simulink model "oc_exm_counter"  (Simulink 6.5)
settings: Solver=FixedStepDiscrete  StartTime=0.0  StopTime=10.0  FixedStep=0.001  RelTol=1e-3
libraries: dsPICdrivers x9
settings Model: Creator=Peter  LastModifiedBy=peter  ProdHWDeviceType=16-bit Generic
settings SolverCC: PositivePriorityOrder=on
settings OptimizationCC: OptimizeModelRefInitCode=on  LifeSpan=1
settings HardwareCC: ProdBitPerInt=16  ProdEndianess=LittleEndian  ProdWordSize=16  ProdHWDeviceType=16-bit Generic  TargetHWDeviceType=32-bit Generic
settings RTWCC: SystemTargetFile=dspic.tlc  TemplateMakefile=dspic_pic30_gcc.tmf  PostCodeGenCommand=dsPIC_Compile()  Description=Embedded Target for Microchip dsPIC (real-time)  ProcessScript=dspic_make_rtw_hook
settings CodeAppCC: IgnoreCustomStorageClasses=off
settings STFCustomTargetCC: TargetFcnLib=ansi_tfl_tmw.mat  GenFloatMathFcnCalls=ANSI_C  ModelReferenceCompliant=off  IncludeMdlTerminateFcn=off  CombineOutputUpdateFcns=on  SuppressErrorStatus=on  ERTCustomFileBanners=on  SupportContinuousTime=off  SupportNonInlinedSFcns=off  SystemTargetFile=dspic.tlc
settings ERTTargetCC: TargetFcnLib=ansi_tfl_tmw.mat  GenFloatMathFcnCalls=ANSI_C  ModelReferenceCompliant=off  IncludeMdlTerminateFcn=off  SuppressErrorStatus=on  InlinedParameterPlacement=NonHierarchical  ERTSrcFileBannerTemplate=dsPIC_code_template.cgt  ERTHdrFileBannerTemplate=dsPIC_code_template.cgt  ERTDataSrcFileTemplate=dsPIC_code_template.cgt  ERTDataHdrFileTemplate=dsPIC_code_template.cgt  ERTCustomFileTemplate=dsPIC_main.tlc
settings CustomProperty: DataType=string  Value=C:\MATLAB\R2006b\rtw\bin\win32\gmake

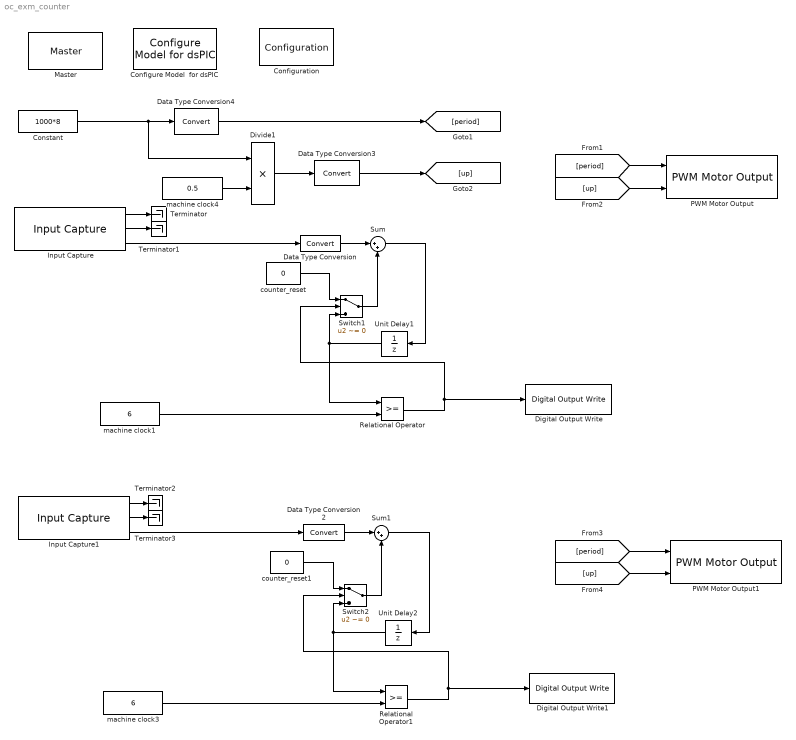
== system oc_exm_counter ==
  Configuration : dsPICdrivers/Configuration  SystemSampleTime=-1  double64=on
  Configure Model  for dsPIC : dsPICdrivers/Simulink Configuration/Configure Model  for dsPIC
  Constant : Constant  Value=1000*8  OutDataTypeMode=double  OutDataType=sfix(16)  ConRadixGroup=Use specified scaling  OutScaling=2^0  SampleTime=-1  FramePeriod=inf
  Data Type Conversion : DataTypeConversion  OutDataTypeMode=double
  Data Type Conversion2 : DataTypeConversion  OutDataTypeMode=double
  Data Type Conversion3 : DataTypeConversion  OutDataTypeMode=uint16
  Data Type Conversion4 : DataTypeConversion  OutDataTypeMode=uint16
  Digital Output Write : dsPICdrivers/Digital I//O/Digital Output Write  Tag=dsPIC_Digital_Output  Priority=5  PORT=E  Pin=[3]  Simultaneous=off  OrderingInOutPopup=None
  Digital Output Write1 : dsPICdrivers/Digital I//O/Digital Output Write  Tag=dsPIC_Digital_Output  Priority=5  PORT=E  Pin=[5]  Simultaneous=off  OrderingInOutPopup=None
  Divide1 : Product  Inputs=**  OutDataTypeMode=double  OutDataType=ufix(16)  OutScaling=2^-1  SaturateOnIntegerOverflow=on
  Input Capture : dsPICdrivers/Peripheral I//O/Input Capture  Tag=dsPIC_PWM_IC  Priority=5  IntPriority=4  Channel=[ 2 ]  Channel_UP_Down_Periode=[5]  MaxChannel=[0.001]  SafeMarge=[10]  MaxName=' IC2max '  Precision=[13.103]  Timer=[2]  ChangeDetected=[2]  ChangeDetectedPortRef=3  SampleTime=-1  Status=OK
  Input Capture1 : dsPICdrivers/Peripheral I//O/Input Capture  Tag=dsPIC_PWM_IC  Priority=5  IntPriority=6  Channel=[1]  Channel_UP_Down_Periode=[5]  MaxChannel=[0.001]  SafeMarge=[10]  MaxName=' IC1max '  Precision=[13.103]  Timer=[2]  ChangeDetected=[2]  ChangeDetectedPortRef=3  SampleTime=-1  Status=OK
  Master : dsPICdrivers/Master  Tag=dsPIC_MASTER  Priority=1  TimeStepType=Timer1  picType=30f4011  fcy=8e6  Quartz_33f=5e6  PLLActive_33f=off  fcyDesired_33f=0  tmr1="[1  7999  0]"  tmr1Info="Time Step : 0.001  ;   Error : 0%  PR1=7999"  tmr2345="[1  0  0  0]"  tmr2345cfg=[-1 -1 -1 -1]  IOautoConf=on  typePort="[ 0   0   0   0   0   0   0   0   0   0   0   0   0   0   0   0   0   0   0   0   6   6   0   0   0   0   0   0   0   0   0   0   0   0   0   0   0   0   0   0   0   0   0   0   0   0   0   0   0   0   0   0   0   0   0   0   0   0   0   0   0   0   0   0  11   0  11  10   0  10   0   0   0   0   0   0   0   0   0   0   0   0   0   0   0   0   0   0   0   0   0   0   0   0   0   0   0   0   0   0   0   0   0   0   0   0   0   0   0   0   0   0 ]"  TRIS="[ 65535  65535  65535  65535  65495  65535  65535 ]"  ADPCFG=48  MasterBusyPort=None  MasterOverloadPort=None  FOSC=FRC_PLL8  ClockSwitchMonitor=Both disabled  TempProtection_33f=TEMP_ON  FPBOR=PBOR_OFF  PWRT=PWRT_4  MCLR=MCLR_DIS  PowerSave=off  OverrideFcy=off  NewFcy=1e6  PR2345="[65535  65535  65535  65535]"
  PWM Motor Output : dsPICdrivers/Peripheral I//O/PWM Motor Output  Tag=dsPIC_PWM_Motor  Priority=5  InputEnableChk=off  InputPeriodeChk=on  Channel=[1 ]  TPeriode=.001  PrescalerValue=1  PeriodeInteger=8000  MaxName='PWM'  Centered=off  HChannelON=off  Info="Nbr Bits : 13.9658  ||  PWM = 16000  ||  Prescaler = 1"  Delay=0  IntPriority=5  nbrPwmChannelPIC=3  Status=OK
  PWM Motor Output1 : dsPICdrivers/Peripheral I//O/PWM Motor Output  Tag=dsPIC_PWM_Motor  Priority=5  InputEnableChk=off  InputPeriodeChk=on  Channel=[2]  TPeriode=.001  PrescalerValue=1  PeriodeInteger=8000  MaxName='PWM'  Centered=off  HChannelON=off  Info="Nbr Bits : 13.9658  ||  PWM = 16000  ||  Prescaler = 1"  Delay=0  IntPriority=5  nbrPwmChannelPIC=3  Status=OK
  Relational Operator : RelationalOperator  LogicOutDataTypeMode=Boolean
  Relational Operator1 : RelationalOperator  LogicOutDataTypeMode=Boolean
  Sum : Sum  Inputs=|++
  Sum1 : Sum  Inputs=|++
  Switch1 : Switch  Criteria=u2 ~= 0
  Switch2 : Switch  Criteria=u2 ~= 0
  Terminator{,1..3} (4 alike) : Terminator
  Unit Delay1 : UnitDelay  Orientation=left  SampleTime=-1
  Unit Delay2 : UnitDelay  Orientation=left  SampleTime=-1
  counter_reset : Constant  Value=0  OutDataTypeMode=double  OutDataType=sfix(16)  ConRadixGroup=Use specified scaling  OutScaling=2^-2  SampleTime=inf  FramePeriod=inf
  counter_reset1 : Constant  Value=0  OutDataTypeMode=double  OutDataType=sfix(16)  ConRadixGroup=Use specified scaling  OutScaling=2^-2  SampleTime=inf  FramePeriod=inf
  machine clock1 : Constant  Value=6  OutDataTypeMode=double  OutDataType=sfix(16)  ConRadixGroup=Use specified scaling  OutScaling=2^-2  SampleTime=inf  FramePeriod=inf
  machine clock3 : Constant  Value=6  OutDataTypeMode=double  OutDataType=sfix(16)  ConRadixGroup=Use specified scaling  OutScaling=2^-2  SampleTime=inf  FramePeriod=inf
  machine clock4 : Constant  Value=0.5  OutDataTypeMode=double  OutDataType=sfix(16)  ConRadixGroup=Use specified scaling  OutScaling=2^-2  SampleTime=inf  FramePeriod=inf
  wires:
  Constant/1 -> Data Type Conversion4/1, Divide1/1
  Data Type Conversion4/1 -> [period]
  Input Capture/3 -> Data Type Conversion/1
  counter_reset/1 -> Switch1/1
  Switch1/1 -> Sum/2
  machine clock1/1 -> Relational Operator/2
  Sum/1 -> Unit Delay1/1
  Unit Delay1/1 -> Relational Operator/1, Switch1/3
  Data Type Conversion/1 -> Sum/1
  Relational Operator/1 -> Switch1/2, Digital Output Write/1
  [period] -> PWM Motor Output/1
  machine clock4/1 -> Divide1/2
  Divide1/1 -> Data Type Conversion3/1
  Data Type Conversion3/1 -> [up]
  [up] -> PWM Motor Output/2
  Input Capture1/3 -> Data Type Conversion2/1
  counter_reset1/1 -> Switch2/1
  Switch2/1 -> Sum1/2
  machine clock3/1 -> Relational Operator1/2
  Sum1/1 -> Unit Delay2/1
  Unit Delay2/1 -> Switch2/3, Relational Operator1/1
  Data Type Conversion2/1 -> Sum1/1
  Relational Operator1/1 -> Switch2/2, Digital Output Write1/1
  [up] -> PWM Motor Output1/2
  [period] -> PWM Motor Output1/1
  Input Capture/1 -> Terminator/1
  Input Capture/2 -> Terminator1/1
  Input Capture1/1 -> Terminator2/1
  Input Capture1/2 -> Terminator3/1
